simulink model "DAB_waveform_model"  (R2022b)
settings: Solver=VariableStepAuto  StartTime=0.0  StopTime=0.3  RelTol=1e-3
undefined symbols (not defined in the file): C_bulk_h, C_bulk_l, f_sw_curr, inductor, L_cab_h, L_cab_l, R_cab_h, R_cab_l, source, T, trans
libraries: spsMosfetLib x8, spsSeriesRLCBranchLib x8, spsCurrentMeasurementLib x3, spsVoltageMeasurementLib x3, spsDCVoltageSourceLib x2, spsLinearTransformerLib x1, slpidlib x1, spspowerguiLib x1
settings Model: Creator=SURFACE  LastModifiedBy=SURFACE

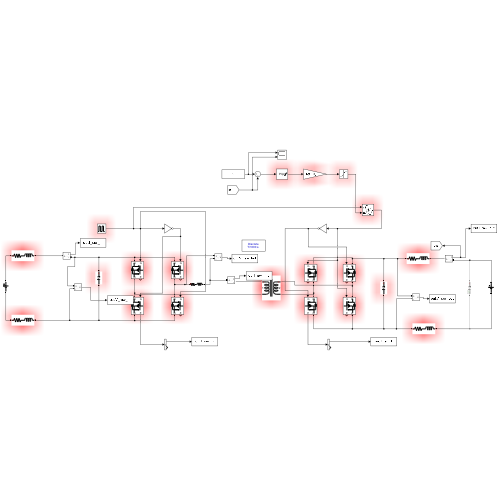
[thumbnail: Simulink's stored preview of the top-level diagram]
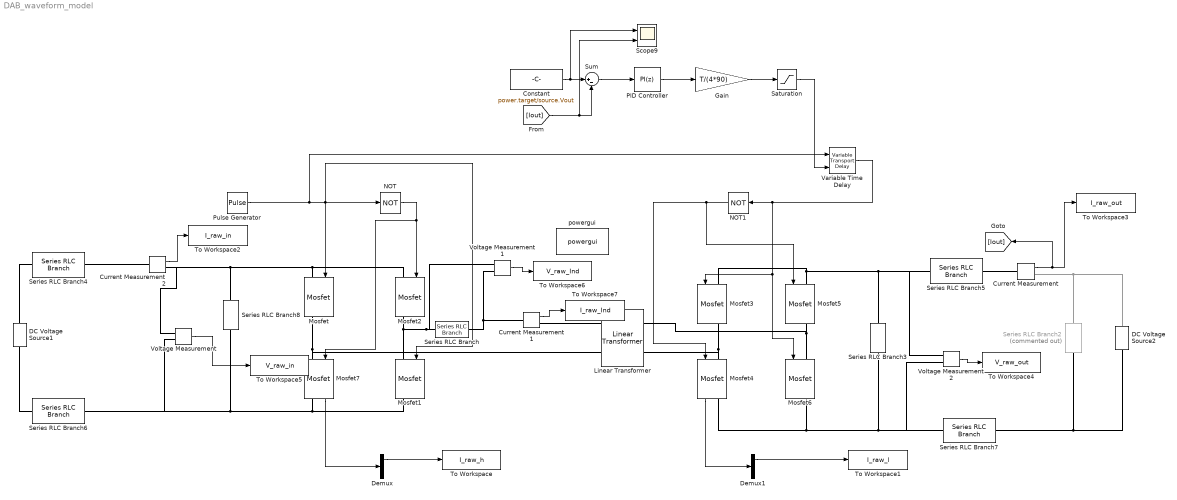
== system DAB_waveform_model ==
  Constant : Constant  Value=power.target/source.Vout
  Current Measurement : spsCurrentMeasurementLib/Current Measurement  PhasorSimulation=off  OutputType=Complex  PSBequivalent=0
  Current Measurement1 : spsCurrentMeasurementLib/Current Measurement  PhasorSimulation=off  OutputType=Complex  PSBequivalent=0
  Current Measurement2 : spsCurrentMeasurementLib/Current Measurement  PhasorSimulation=off  OutputType=Complex  PSBequivalent=0
  DC Voltage Source1 : spsDCVoltageSourceLib/DC Voltage Source  Amplitude=source.Vin  Measurements=None
  DC Voltage Source2 : spsDCVoltageSourceLib/DC Voltage Source  Amplitude=source.Vout  Measurements=None
  Demux : Demux  Outputs=2
      settings: DisplayOption=none
  Demux1 : Demux  Outputs=2
      settings: DisplayOption=none
  Gain : Gain  Gain=T/(4*90)
  Linear Transformer : spsLinearTransformerLib/Linear Transformer  UNITS=SI  NominalPower=[trans.power f_sw_curr ]  winding1=[trans.V1 trans.R1 0]  winding2=[trans.V2 trans.R2 0]  ThreeWindings=off  winding3=[3.15e+05 198.45 1.2634]  RmLm=[trans.Rm trans.Lm]  Measurements=None  DataType=on
  Mosfet{,1..2,7} (4 alike) : spsMosfetLib/Mosfet  Ron=R_on_h  Lon=0  Rd=R_d_h  Vfd=V_f_h  IC=0  Rs=R_s  Cs=inf  Measurements=on
  Mosfet{3..6} (4 alike) : spsMosfetLib/Mosfet  Ron=R_on_l  Lon=0  Rd=R_d_l  Vfd=V_f_l  IC=0  Rs=R_s  Cs=inf  Measurements=on
  NOT : Logic  Operator=NOT  IconShape=distinctive  AllPortsSameDT=off  OutDataTypeStr=boolean
  NOT1 : Logic  Operator=NOT  IconShape=distinctive  AllPortsSameDT=off  OutDataTypeStr=boolean
  PID Controller : slpidlib/PID Controller  Controller=PI  Form=Parallel  TimeDomain=Discrete-time  UseExternalTs=off  SampleTime=T/1000  IntegratorMethod=Forward Euler  FilterMethod=Forward Euler  ControllerParametersSource=internal  P=90/(power.target/source.Vout)  I=90/(power.target/source.Vout)*50  UseKiTs=off  D=0  N=100  UseFilter=on  TunerSelectOption=Transfer Function Based (PID Tuner App)  InitialConditionSource=internal  InitialConditionForIntegrator=0  InitialConditionForFilter=0  DifferentiatorICPrevScaledInput=0  ExternalReset=none  TrackingMode=off  Kt=1  LimitOutput=on  SatLimitsSource=internal  UpperSaturationLimit=80  LowerSaturationLimit=-80  LinearizeAsGain=on  AntiWindupMode=none  Kb=1  LimitIntegrator=off  UpperIntegratorSaturationLimit=inf  LowerIntegratorSaturationLimit=-inf  POutMin=[]  POutMax=[]  IOutMin=[]  IOutMax=[]  DOutMin=[]  DOutMax=[]  NOutMin=[]  NOutMax=[]  SumOutMin=[]  SumOutMax=[]  SaturationOutMin=[]  SaturationOutMax=[]  PParamMin=[]  PParamMax=[]  IParamMin=[]  IParamMax=[]  DParamMin=[]  DParamMax=[]  NParamMin=[]  NParamMax=[]  KbParamMin=[]  KbParamMax=[]  KtParamMin=[]  KtParamMax=[]  KbOutMin=[]  KbOutMax=[]  KtOutMin=[]  KtOutMax=[]  IntegratorOutMin=[]  IntegratorOutMax=[]  FilterOutMin=[]  FilterOutMax=[]  SumI1OutMin=[]  SumI1OutMax=[]  SumI2OutMin=[]  SumI2OutMax=[]  SumI3OutMin=[]  SumI3OutMax=[]  SumI4OutMin=[]  SumI4OutMax=[]  SumDOutMin=[]  SumDOutMax=[]  DifferentiatorOutMin=[]  DifferentiatorOutMax=[]  FilterDiffOutCoefMin=[]  FilterDiffOutCoefMax=[]  ReciprocalOutMin=[]  ReciprocalOutMax=[]  SumDenOutMin=[]  SumDenOutMax=[]  SumNumOutMin=[]  SumNumOutMax=[]  DivideOutMin=[]  DivideOutMax=[]  UdiffTsProdOutMin=[]  UdiffTsProdOutMax=[]  NTsProdOutMin=[]  NTsProdOutMax=[]  UintegralTsProdOutMin=[]  UintegralTsProdOutMax=[]  UngainTsProdOutMin=[]  UngainTsProdOutMax=[]  ClampingZeroOutDataTypeStr=Inherit: Inherit via back propagation  ClampingZeroOutMin=[]  ClampingZeroOutMax=[]  FilterDenConstantOutDataTypeStr=Inherit: Inherit via back propagation  FilterDenConstantOutMin=[]  FilterDenConstantOutMax=[]  PCopyOutDataTypeStr=Inherit: Inherit via back propagation  PCopyOutMin=[]  PCopyOutMax=[]  NCopyOutDataTypeStr=Inherit: Inherit via back propagation  NCopyOutMin=[]  NCopyOutMax=[]  IntegratorContinuousStateAttributes=''  IntegratorStateMustResolveToSignalObject=off  IntegratorRTWStateStorageClass=Auto  FilterContinuousStateAttributes=''  FilterStateMustResolveToSignalObject=off  FilterRTWStateStorageClass=Auto  ParallelPVariant=InternalParameters  IdealPVariant=Disabled  IVariant=InternalParameters  DVariant=Disabled  IntegratorVariant=Discrete  SatVariant=Enabled  AWVariant=Passthrough  PCopyVariant=Disabled  TRVariant=Disabled  FdbkBlocksVariant=Forward  IdealPFdbkVariant=Disabled  SatFdbkVariant=Disabled  DerivativeFilterVariant=Disabled  NVariant=Disabled  NCopyVariant=Disabled_SignalSpec  FilterICVariant=Disabled  IntegratorICVariant=InternalICs  ExternalResetVariant=Disabled  TRSumVariant=Passthrough  SumFdbkVariant=Disabled  SumVariant=Sum_PI  TsampFilterVariant=InternalTs  TsampNgainVariant=Passthrough  TsampIntegralVariant=Passthrough  ExternalSaturationOutDataTypeStr=Inherit: Same as second input
  Pulse Generator : DiscretePulseGenerator  PulseType=Time based  Period=T  PulseWidth=50
  Saturation : Saturate  UpperLimit=inf  LowerLimit=T/1000
  Scope9 : Scope  NumInputPorts=2
  Series RLC Branch : spsSeriesRLCBranchLib/Series RLC Branch  LConnTagsString=__new0  RConnTagsString=__new0  BranchType=RL  Resistance=inductor.Rdc  Inductance=inductor.Lk  SetiL0=off  InitialCurrent=0  Capacitance=1e-6  Setx0=off  InitialVoltage=0  Measurements=Branch voltage and current
  Series RLC Branch2 : spsSeriesRLCBranchLib/Series RLC Branch  Commented=on  LConnTagsString=__new0  RConnTagsString=__new0  BranchType=C  Resistance=1  Inductance=.5e-5  SetiL0=off  InitialCurrent=0  Capacitance=3e-5  Setx0=off  InitialVoltage=0  Measurements=None
  Series RLC Branch3 : spsSeriesRLCBranchLib/Series RLC Branch  LConnTagsString=__new0  RConnTagsString=__new0  BranchType=C  Resistance=1  Inductance=.5e-5  SetiL0=off  InitialCurrent=0  Capacitance=C_bulk_l  Setx0=off  InitialVoltage=0  Measurements=None
  Series RLC Branch4 : spsSeriesRLCBranchLib/Series RLC Branch  LConnTagsString=__new0  RConnTagsString=__new0  BranchType=RL  Resistance=R_cab_h  Inductance=L_cab_h  SetiL0=off  InitialCurrent=0  Capacitance=1.8e-9  Setx0=off  InitialVoltage=0  Measurements=None
  Series RLC Branch5 : spsSeriesRLCBranchLib/Series RLC Branch  LConnTagsString=__new0  RConnTagsString=__new0  BranchType=RL  Resistance=R_cab_l  Inductance=L_cab_l  SetiL0=off  InitialCurrent=0  Capacitance=1.8e-9  Setx0=off  InitialVoltage=0  Measurements=None
  Series RLC Branch6 : spsSeriesRLCBranchLib/Series RLC Branch  LConnTagsString=__new0  RConnTagsString=__new0  BranchType=RL  Resistance=R_cab_h  Inductance=L_cab_h  SetiL0=off  InitialCurrent=0  Capacitance=1.8e-9  Setx0=off  InitialVoltage=0  Measurements=None
  Series RLC Branch7 : spsSeriesRLCBranchLib/Series RLC Branch  LConnTagsString=__new0  RConnTagsString=__new0  BranchType=RL  Resistance=R_cab_l  Inductance=L_cab_l  SetiL0=off  InitialCurrent=0  Capacitance=1.8e-9  Setx0=off  InitialVoltage=0  Measurements=None
  Series RLC Branch8 : spsSeriesRLCBranchLib/Series RLC Branch  LConnTagsString=__new0  RConnTagsString=__new0  BranchType=C  Resistance=1  Inductance=.5e-5  SetiL0=off  InitialCurrent=0  Capacitance=C_bulk_h  Setx0=off  InitialVoltage=0  Measurements=None
  Sum : Sum  Inputs=|+-
  To Workspace : ToWorkspace  VariableName=I_raw_h  SaveFormat=Timeseries  SampleTime=-1
  To Workspace1 : ToWorkspace  VariableName=I_raw_l  SaveFormat=Timeseries  SampleTime=-1
  To Workspace2 : ToWorkspace  VariableName=I_raw_in  SaveFormat=Timeseries  SampleTime=-1
  To Workspace3 : ToWorkspace  VariableName=I_raw_out  SaveFormat=Timeseries  SampleTime=-1
  To Workspace4 : ToWorkspace  VariableName=V_raw_out  SaveFormat=Timeseries  SampleTime=-1
  To Workspace5 : ToWorkspace  VariableName=V_raw_in  SaveFormat=Timeseries  SampleTime=-1
  To Workspace6 : ToWorkspace  VariableName=V_raw_Ind  SaveFormat=Timeseries  SampleTime=-1
  To Workspace7 : ToWorkspace  VariableName=I_raw_Ind  SaveFormat=Timeseries  SampleTime=-1
  Variable Time Delay : VariableTransportDelay  MaximumDelay=T  ZeroDelay=on
  Voltage Measurement : spsVoltageMeasurementLib/Voltage Measurement  PhasorSimulation=off  OutputType=Complex  PSBequivalent=0
  Voltage Measurement1 : spsVoltageMeasurementLib/Voltage Measurement  PhasorSimulation=off  OutputType=Complex  PSBequivalent=0
  Voltage Measurement2 : spsVoltageMeasurementLib/Voltage Measurement  PhasorSimulation=off  OutputType=Complex  PSBequivalent=0
  powergui : spspowerguiLib/powergui  Priority=1  SimulationMode=Discrete  SampleTime=T/1000  frequency=60  Iterations=50  frequencyindice=0  Pbase=100e6  ErrMax=1e-4  UnitsV=kV  UnitsW=MW  buscounter=0  FunctionMessages=off  echomessages=off  EnableUseOfTLC=off  CurrentSourceSwitches=off  DisableSnubberDevices=off  DisableRonSwitches=off  DisableVfSwitches=off  DisplayEquations=off  AutomaticDiscreteSolvers=off  SolverType=Tustin/Backward Euler (TBE)  Interpol=off  ExternalGateDelay=off  methode=off  Ts=100  x0status=blocks  SPID=on  SwTol=0  HookPort=off  NonlinearTolerance=1e-4  nMaxIteration=100  ContinueOnMaxIteration=off  RestoreLinks=warning  ResistiveCurrentMeasurement=off  Frange=[0:2:500]  Ylog=off  Xlog=on  ShowGrid=off  save=off  variable=ZData  structure=0  ZoomFFT=off  StartTime=0.0  cycles=1  DisplayStyle=1  fundamental=60  FreqAxis=off  MaxFrequency=1000  frequencyindicesteady=1  RmsSteady=1  display=off
  wires:
  Pulse Generator/1 -> Variable Time Delay/1, Mosfet1/1, NOT/1, Mosfet/1
  NOT/1 -> Mosfet2/1, Mosfet7/1
  Variable Time Delay/1 -> Mosfet6/1, Mosfet3/1, NOT1/1
  NOT1/1 -> Mosfet5/1, Mosfet4/1
  Gain/1 -> Saturation/1
  Mosfet7/1 -> Demux/1
  Demux/1 -> To Workspace/1
  Demux1/1 -> To Workspace1/1
  Mosfet4/1 -> Demux1/1
  Current Measurement2/1 -> To Workspace2/1
  Current Measurement/1 -> [Iout], To Workspace3/1
  Constant/1 -> Scope9/1, Sum/1
  [Iout] -> Scope9/2, Sum/2
  Sum/1 -> PID Controller/1
  PID Controller/1 -> Gain/1
  Saturation/1 -> Variable Time Delay/2
  Voltage Measurement2/1 -> To Workspace4/1
  Voltage Measurement/1 -> To Workspace5/1
  Voltage Measurement1/1 -> To Workspace6/1
  Current Measurement1/1 -> To Workspace7/1
  connections:
  Voltage Measurement/LConn2 -- Series RLC Branch6/RConn1 -- Series RLC Branch8/RConn1 -- Mosfet1/RConn1 -- Mosfet7/RConn1
  Mosfet7/LConn1 -- Mosfet/RConn1 -- Linear Transformer/LConn2
  Series RLC Branch/LConn1 -- Mosfet2/RConn1 -- Mosfet1/LConn1 -- Voltage Measurement1/LConn1
  Voltage Measurement1/LConn2 -- Series RLC Branch/RConn1 -- Current Measurement1/LConn1
  Linear Transformer/RConn2 -- Mosfet3/RConn1 -- Mosfet4/LConn1
  Voltage Measurement2/LConn2 -- Series RLC Branch7/LConn1 -- Series RLC Branch3/RConn1 -- Mosfet4/RConn1 -- Mosfet6/RConn1
  Linear Transformer/RConn1 -- Mosfet5/RConn1 -- Mosfet6/LConn1
  Current Measurement2/LConn1 -- Series RLC Branch4/RConn1
  Series RLC Branch4/LConn1 -- DC Voltage Source1/RConn1
  Series RLC Branch6/LConn1 -- DC Voltage Source1/LConn1
  Series RLC Branch7/RConn1 -- DC Voltage Source2/LConn1 -- Series RLC Branch2/RConn1
  Series RLC Branch2/LConn1 -- DC Voltage Source2/RConn1 -- Current Measurement/RConn1
  Series RLC Branch5/RConn1 -- Current Measurement/LConn1
  Mosfet3/LConn1 -- Voltage Measurement2/LConn1 -- Series RLC Branch5/LConn1 -- Series RLC Branch3/LConn1 -- Mosfet5/LConn1
  Mosfet/LConn1 -- Mosfet2/LConn1 -- Voltage Measurement/LConn1 -- Current Measurement2/RConn1 -- Series RLC Branch8/LConn1
  Current Measurement1/RConn1 -- Linear Transformer/LConn1
